simulink model "ASM_Traffic"  (R2026a)
settings: Solver=ode1  StartTime=SIM.tstart.v  StopTime=SIM.tend.v  FixedStep=SIM.StepSize.v
PostLoadFcn:
  | if any(exist('dsrtsu_mdlpostloadfcn', 'file') ~= 0), dsrtsu_mdlpostloadfcn('Execute', bdroot); end
  | try, asm_mdl_postloadfcn(bdroot, 'UpdateModel', 3600); catch, disp(lasterr); end,
InitFcn:
  | , if any(exist('rtifpga_mdlclblib', 'file') ~= 0), rtifpga_mdlclblib('Init', bdroot); end,
  | , if any(exist('dsmpb_private', 'file') ~= 0), dsmpb_private('dsmpb_mdlclblib', 'Init', bdroot); end,
model workspace (MAT data in the model file):
  asmReferencePath = [0 0.01 0.02 0.03 0.04 0.05 0.06 0.07 0.08 0.09 0.1 0.11 ... (350007 elements, 50001x7)]
  roadBounds : Simulink.Parameter (value not decoded)
  safetyAxes : Simulink.Parameter (value not decoded)
undefined symbols (not defined in the file): _to_, a0b2, ASM_BrakeHydraulics_DemoSystems, ASM_VehicleDynamics_DemoSystems, b98103fe8ad365046cd0, BrakeCircuit, controllerConfig, CPT, Crankshaft, DiscIntNeverNeededParam, dsmsi, FinalDriveAssembly, MDL, ModeSignals, mu, Pos_BrakePedal_Maneuver, rad, RefSignals, roadFamilyData, roadFamilyId, s_to_rpm, SIM, SoftECU, Suspension, Tire, Transmission
libraries: ASM_Traffic_lib x135, simulink x98, ASM_Utils_lib x77, ASM_VehicleDynamics_lib x70, ASM_Environment_lib x22, dsmpblib x20, dsmsilib x15, MDLD_Utils_lib x10, ASM_BrakeHydraulics_lib x3, sl_discontinuities x2
(part 49 of 65)

== system ASM_Traffic/Environment/Road/UserInterface/PAR_Plant/Objects_DataStreams/DataStream_5 ==
  Maneuver_Signals[] : Inport
  Bus Creator1 : BusCreator  Inputs=5
  Bus Selector2 : BusSelector  OutputSignals=Mnv_DataStream_5[]
  Ext_DataStream_5[] : Constant  Value=0
  Multiport Switch : MultiPortSwitch  DataPortOrder=Zero-based contiguous  zeroidx=on  SaturateOnIntegerOverflow=off  InputSameDT=off
  Rounding Function : Rounding  Operator=round
  Saturation : Saturate  UpperLimit=2  LowerLimit=0
  Stim_DataStream_5[] : Constant  Value=0
  Sw_DataStream_5[0Stim|1Ext|2Mnv] : Constant  Value=2
  avoid_incomplete_trace2source : Subsystem
  DataStream_5[] : Outport  VectorParamsAs1DForOutWhenUnconnected=off
  wires:
  avoid_incomplete_trace2source/1(Out1) -> Bus Creator1/3  "Mnv_DataStream_5[]"
  Sw_DataStream_5[0Stim|1Ext|2Mnv]/1 -> Rounding Function/1, Bus Creator1/1  "Sw_DataStream_5[0Stim|1Ext|2Mnv]"
  Maneuver_Signals[]/1 -> Bus Selector2/1
  Ext_DataStream_5[]/1 -> Multiport Switch/3, Bus Creator1/4  "Ext_DataStream_5[]"
  Bus Selector2/1 -> Multiport Switch/4, avoid_incomplete_trace2source/1(In1)  "<Mnv_DataStream_5[]>"
  Rounding Function/1 -> Saturation/1
  Saturation/1 -> Multiport Switch/1
  Multiport Switch/1 -> Bus Creator1/5  "DataStream_5[]"
  Stim_DataStream_5[]/1 -> Multiport Switch/2, Bus Creator1/2  "Stim_DataStream_5[]"
  Bus Creator1/1 -> DataStream_5[]/1

== system ASM_Traffic/Environment/Road/UserInterface/PAR_Plant/Objects_DataStreams/DataStream_6 ==
  Maneuver_Signals[] : Inport
  Bus Creator1 : BusCreator  Inputs=5
  Bus Selector2 : BusSelector  OutputSignals=Mnv_DataStream_6[]
  Ext_DataStream_6[] : Constant  Value=0
  Multiport Switch : MultiPortSwitch  DataPortOrder=Zero-based contiguous  zeroidx=on  SaturateOnIntegerOverflow=off  InputSameDT=off
  Rounding Function : Rounding  Operator=round
  Saturation : Saturate  UpperLimit=2  LowerLimit=0
  Stim_DataStream_6[] : Constant  Value=0
  Sw_DataStream_6[0Stim|1Ext|2Mnv] : Constant  Value=2
  avoid_incomplete_trace2source : Subsystem
  DataStream_6[] : Outport  VectorParamsAs1DForOutWhenUnconnected=off
  wires:
  avoid_incomplete_trace2source/1(Out1) -> Bus Creator1/3  "Mnv_DataStream_6[]"
  Bus Creator1/1 -> DataStream_6[]/1
  Stim_DataStream_6[]/1 -> Bus Creator1/2, Multiport Switch/2  "Stim_DataStream_6[]"
  Multiport Switch/1 -> Bus Creator1/5  "DataStream_6[]"
  Saturation/1 -> Multiport Switch/1
  Rounding Function/1 -> Saturation/1
  Bus Selector2/1 -> Multiport Switch/4, avoid_incomplete_trace2source/1(In1)  "<Mnv_DataStream_6[]>"
  Ext_DataStream_6[]/1 -> Multiport Switch/3, Bus Creator1/4  "Ext_DataStream_6[]"
  Maneuver_Signals[]/1 -> Bus Selector2/1
  Sw_DataStream_6[0Stim|1Ext|2Mnv]/1 -> Bus Creator1/1, Rounding Function/1  "Sw_DataStream_6[0Stim|1Ext|2Mnv]"

== system ASM_Traffic/Environment/Road/UserInterface/PAR_Plant/Objects_DataStreams/DataStream_7 ==
  Maneuver_Signals[] : Inport
  Bus Creator1 : BusCreator  Inputs=5
  Bus Selector2 : BusSelector  OutputSignals=Mnv_DataStream_7[]
  Ext_DataStream_7[] : Constant  Value=0
  Multiport Switch : MultiPortSwitch  DataPortOrder=Zero-based contiguous  zeroidx=on  SaturateOnIntegerOverflow=off  InputSameDT=off
  Rounding Function : Rounding  Operator=round
  Saturation : Saturate  UpperLimit=2  LowerLimit=0
  Stim_DataStream_7[] : Constant  Value=0
  Sw_DataStream_7[0Stim|1Ext|2Mnv] : Constant  Value=2
  avoid_incomplete_trace2source : Subsystem
  DataStream_7[] : Outport  VectorParamsAs1DForOutWhenUnconnected=off
  wires:
  avoid_incomplete_trace2source/1(Out1) -> Bus Creator1/3  "Mnv_DataStream_7[]"
  Sw_DataStream_7[0Stim|1Ext|2Mnv]/1 -> Rounding Function/1, Bus Creator1/1  "Sw_DataStream_7[0Stim|1Ext|2Mnv]"
  Maneuver_Signals[]/1 -> Bus Selector2/1
  Ext_DataStream_7[]/1 -> Multiport Switch/3, Bus Creator1/4  "Ext_DataStream_7[]"
  Bus Selector2/1 -> Multiport Switch/4, avoid_incomplete_trace2source/1(In1)  "<Mnv_DataStream_7[]>"
  Rounding Function/1 -> Saturation/1
  Saturation/1 -> Multiport Switch/1
  Multiport Switch/1 -> Bus Creator1/5  "DataStream_7[]"
  Stim_DataStream_7[]/1 -> Multiport Switch/2, Bus Creator1/2  "Stim_DataStream_7[]"
  Bus Creator1/1 -> DataStream_7[]/1

== system ASM_Traffic/Environment/Road/UserInterface/PAR_Plant/Objects_DataStreams/DataStream_8 ==
  Maneuver_Signals[] : Inport
  Bus Creator1 : BusCreator  Inputs=5
  Bus Selector2 : BusSelector  OutputSignals=Mnv_DataStream_8[]
  Ext_DataStream_8[] : Constant  Value=0
  Multiport Switch : MultiPortSwitch  DataPortOrder=Zero-based contiguous  zeroidx=on  SaturateOnIntegerOverflow=off  InputSameDT=off
  Rounding Function : Rounding  Operator=round
  Saturation : Saturate  UpperLimit=2  LowerLimit=0
  Stim_DataStream_8[] : Constant  Value=0
  Sw_DataStream_8[0Stim|1Ext|2Mnv] : Constant  Value=2
  avoid_incomplete_trace2source : Subsystem
  DataStream_8[] : Outport  VectorParamsAs1DForOutWhenUnconnected=off
  wires:
  avoid_incomplete_trace2source/1(Out1) -> Bus Creator1/3  "Mnv_DataStream_8[]"
  Bus Creator1/1 -> DataStream_8[]/1
  Stim_DataStream_8[]/1 -> Bus Creator1/2, Multiport Switch/2  "Stim_DataStream_8[]"
  Multiport Switch/1 -> Bus Creator1/5  "DataStream_8[]"
  Saturation/1 -> Multiport Switch/1
  Rounding Function/1 -> Saturation/1
  Bus Selector2/1 -> Multiport Switch/4, avoid_incomplete_trace2source/1(In1)  "<Mnv_DataStream_8[]>"
  Ext_DataStream_8[]/1 -> Multiport Switch/3, Bus Creator1/4  "Ext_DataStream_8[]"
  Maneuver_Signals[]/1 -> Bus Selector2/1
  Sw_DataStream_8[0Stim|1Ext|2Mnv]/1 -> Bus Creator1/1, Rounding Function/1  "Sw_DataStream_8[0Stim|1Ext|2Mnv]"

== system ASM_Traffic/Environment/Sensors/PlantModel/Object_Sensor_2D/ASMSignalCollector/Rename ==
  In1 : Inport
  Out1 : Outport  VectorParamsAs1DForOutWhenUnconnected=off
  wires:
  In1/1 -> Out1/1

== system ASM_Traffic/Environment/Sensors/PlantModel/Object_Sensor_2D/ASMSignalCollector/Rename1 ==
  In1 : Inport
  Out1 : Outport  VectorParamsAs1DForOutWhenUnconnected=off
  wires:
  In1/1 -> Out1/1

== system ASM_Traffic/Environment/Sensors/PlantModel/Object_Sensor_2D/ASMSignalCollector/Rename10 ==
  In1 : Inport
  Out1 : Outport  VectorParamsAs1DForOutWhenUnconnected=off
  wires:
  In1/1 -> Out1/1

== system ASM_Traffic/Environment/Sensors/PlantModel/Object_Sensor_2D/ASMSignalCollector/Rename11 ==
  In1 : Inport
  Out1 : Outport  VectorParamsAs1DForOutWhenUnconnected=off
  wires:
  In1/1 -> Out1/1

== system ASM_Traffic/Environment/Sensors/PlantModel/Object_Sensor_2D/ASMSignalCollector/Rename12 ==
  In1 : Inport
  Out1 : Outport  VectorParamsAs1DForOutWhenUnconnected=off
  wires:
  In1/1 -> Out1/1

== system ASM_Traffic/Environment/Sensors/PlantModel/Object_Sensor_2D/ASMSignalCollector/Rename13 ==
  In1 : Inport
  Out1 : Outport  VectorParamsAs1DForOutWhenUnconnected=off
  wires:
  In1/1 -> Out1/1

== system ASM_Traffic/Environment/Sensors/PlantModel/Object_Sensor_2D/ASMSignalCollector/Rename2 ==
  In1 : Inport
  Out1 : Outport  VectorParamsAs1DForOutWhenUnconnected=off
  wires:
  In1/1 -> Out1/1

== system ASM_Traffic/Environment/Sensors/PlantModel/Object_Sensor_2D/ASMSignalCollector/Rename3 ==
  In1 : Inport
  Out1 : Outport  VectorParamsAs1DForOutWhenUnconnected=off
  wires:
  In1/1 -> Out1/1

== system ASM_Traffic/Environment/Sensors/PlantModel/Object_Sensor_2D/ASMSignalCollector/Rename4 ==
  In1 : Inport
  Out1 : Outport  VectorParamsAs1DForOutWhenUnconnected=off
  wires:
  In1/1 -> Out1/1

== system ASM_Traffic/Environment/Sensors/PlantModel/Object_Sensor_2D/ASMSignalCollector/Rename5 ==
  In1 : Inport
  Out1 : Outport  VectorParamsAs1DForOutWhenUnconnected=off
  wires:
  In1/1 -> Out1/1

== system ASM_Traffic/Environment/Sensors/PlantModel/Object_Sensor_2D/ASMSignalCollector/Rename6 ==
  In1 : Inport
  Out1 : Outport  VectorParamsAs1DForOutWhenUnconnected=off
  wires:
  In1/1 -> Out1/1

== system ASM_Traffic/Environment/Sensors/PlantModel/Object_Sensor_2D/ASMSignalCollector/Rename7 ==
  In1 : Inport
  Out1 : Outport  VectorParamsAs1DForOutWhenUnconnected=off
  wires:
  In1/1 -> Out1/1

== system ASM_Traffic/Environment/Sensors/PlantModel/Object_Sensor_2D/ASMSignalCollector/Rename8 ==
  In1 : Inport
  Out1 : Outport  VectorParamsAs1DForOutWhenUnconnected=off
  wires:
  In1/1 -> Out1/1

== system ASM_Traffic/Environment/Sensors/PlantModel/Object_Sensor_2D/ASMSignalCollector/Rename9 ==
  In1 : Inport
  Out1 : Outport  VectorParamsAs1DForOutWhenUnconnected=off
  wires:
  In1/1 -> Out1/1

== system ASM_Traffic/Environment/Sensors/PlantModel/Object_Sensor_2D/ObjectData/Sensor1 ==
  Object_ID[] : Inport
  Object_Type[] : Inport  Port=2
  Traffic_Signals : Inport  Port=3
  Road_Signals : Inport  Port=4
  ASMSignalCollector : Subsystem
  Bus Selector4 : BusSelector  OutputSignals=Plant.Road_TrafficFellows.Network_Item_Type_Fellows[],Plant.Road_TrafficFellows.Network_Item_Id_Fellows[],Plant.TrafficObject_Data[]
  Bus Selector5 : BusSelector  OutputSignals=Plant.Traffic_Signals_toEnvironment
  Bus Selector6 : BusSelector  OutputSignals=Plant.ObjectParameters.TrafficObjects.TrafficObject_Type_Data[]
  GetFellowPositionVector : Subsystem
  OBJECT_POSITION : ASM_Traffic_lib/Objects/OBJECT_POSITION  MaxNumFellows=MDL.Traffic.MaxNumFellows  ASMProperties=struct('Name','OBJECT_POSITION','Version','2.0','Library','ASM_Traffic_lib')  ASMInstanceName=object_position  ASMInstanceID=1
  OBJECT_PROPERTIES_BOX : ASM_Traffic_lib/Objects/OBJECT_PROPERTIES_BOX  ASMProperties=struct('Name','OBJECT_PROPERTIES_BOX','Version','2.0','Library','ASM_Traffic_lib')  ASMInstanceName=object_properties_box  ASMInstanceID=1
  Object_Custom_Values : Subsystem
  Terminator : Terminator
  Terminator1 : Terminator
  ASMSignalBus : Outport  VectorParamsAs1DForOutWhenUnconnected=off
  Object_Position[] : Outport  Port=2  VectorParamsAs1DForOutWhenUnconnected=off
  Object_Properties_Box[] : Outport  Port=3  VectorParamsAs1DForOutWhenUnconnected=off
  Object_Custom_Values[] : Outport  Port=4  VectorParamsAs1DForOutWhenUnconnected=off
  wires:
  Bus Selector5/1 -> GetFellowPositionVector/1(<FellowPositions>)  "<Traffic_Signals_toEnvironment>"
  GetFellowPositionVector/2(Angle_Fellows[deg]) -> OBJECT_POSITION/3
  GetFellowPositionVector/1(Pos_Fellows_MainPnt_CoorSys_E[x;y;z][m]) -> OBJECT_POSITION/2
  OBJECT_PROPERTIES_BOX/2 -> Object_Properties_Box[]/1, ASMSignalCollector/2(Object_Properties_Box)
  ASMSignalCollector/1(ASMSignalBus) -> ASMSignalBus/1
  OBJECT_POSITION/2 -> Object_Position[]/1, ASMSignalCollector/1(Object_Positions)
  Object_Custom_Values/1(Object_Custom_Values[]) -> ASMSignalCollector/3(Object_Custom_Values), Object_Custom_Values[]/1  "Object_Custom_Values"
  Bus Selector6/1 -> Object_Custom_Values/2(TrafficObject_Type_Data[]), OBJECT_PROPERTIES_BOX/2  "<TrafficObject_Type_Data[]>"
  Traffic_Signals/1 -> Bus Selector6/1, Bus Selector5/1
  Bus Selector4/3 -> OBJECT_POSITION/6  "<TrafficObject_Data[]>"
  Bus Selector4/2 -> OBJECT_POSITION/5  "<Network_Item_Id_Fellows[]>"
  Bus Selector4/1 -> OBJECT_POSITION/4  "<Network_Item_Type_Fellows[]>"
  Road_Signals/1 -> Bus Selector4/1
  Object_Type[]/1 -> OBJECT_PROPERTIES_BOX/1, Object_Custom_Values/1(TrafficObject_Type[])
  OBJECT_PROPERTIES_BOX/1 -> Terminator1/1
  Object_ID[]/1 -> OBJECT_POSITION/1
  OBJECT_POSITION/1 -> Terminator/1

== system ASM_Traffic/Environment/Sensors/PlantModel/Object_Sensor_2D/ObjectData/Sensor2 ==
  Object_ID[] : Inport
  Object_Type[] : Inport  Port=2
  Traffic_Signals : Inport  Port=3
  Road_Signals : Inport  Port=4
  ASMSignalCollector : Subsystem
  Bus Selector4 : BusSelector  OutputSignals=Plant.Road_TrafficFellows.Network_Item_Type_Fellows[],Plant.Road_TrafficFellows.Network_Item_Id_Fellows[],Plant.TrafficObject_Data[]
  Bus Selector5 : BusSelector  OutputSignals=Plant.Traffic_Signals_toEnvironment
  Bus Selector6 : BusSelector  OutputSignals=Plant.ObjectParameters.TrafficObjects.TrafficObject_Type_Data[]
  GetFellowPositionVector : Subsystem
  OBJECT_POSITION : ASM_Traffic_lib/Objects/OBJECT_POSITION  MaxNumFellows=MDL.Traffic.MaxNumFellows  ASMProperties=struct('Name','OBJECT_POSITION','Version','2.0','Library','ASM_Traffic_lib')  ASMInstanceName=object_position  ASMInstanceID=1
  OBJECT_PROPERTIES_BOX : ASM_Traffic_lib/Objects/OBJECT_PROPERTIES_BOX  ASMProperties=struct('Name','OBJECT_PROPERTIES_BOX','Version','2.0','Library','ASM_Traffic_lib')  ASMInstanceName=object_properties_box  ASMInstanceID=1
  Object_Custom_Values : Subsystem
  Terminator : Terminator
  Terminator1 : Terminator
  ASMSignalBus : Outport  VectorParamsAs1DForOutWhenUnconnected=off
  Object_Position[] : Outport  Port=2  VectorParamsAs1DForOutWhenUnconnected=off
  Object_Properties_Box[] : Outport  Port=3  VectorParamsAs1DForOutWhenUnconnected=off
  Object_Custom_Values[] : Outport  Port=4  VectorParamsAs1DForOutWhenUnconnected=off
  wires:
  GetFellowPositionVector/1(Pos_Fellows_MainPnt_CoorSys_E[x;y;z][m]) -> OBJECT_POSITION/2
  GetFellowPositionVector/2(Angle_Fellows[deg]) -> OBJECT_POSITION/3
  Traffic_Signals/1 -> Bus Selector6/1, Bus Selector5/1
  Bus Selector5/1 -> GetFellowPositionVector/1(<FellowPositions>)  "<Traffic_Signals_toEnvironment>"
  Object_Custom_Values/1(Object_Custom_Values[]) -> Object_Custom_Values[]/1, ASMSignalCollector/3(Object_Custom_Values)  "Object_Custom_Values"
  OBJECT_POSITION/2 -> Object_Position[]/1, ASMSignalCollector/1(Object_Positions)
  OBJECT_PROPERTIES_BOX/2 -> Object_Properties_Box[]/1, ASMSignalCollector/2(Object_Properties_Box)
  ASMSignalCollector/1(ASMSignalBus) -> ASMSignalBus/1
  OBJECT_POSITION/1 -> Terminator/1
  Object_ID[]/1 -> OBJECT_POSITION/1
  OBJECT_PROPERTIES_BOX/1 -> Terminator1/1
  Object_Type[]/1 -> Object_Custom_Values/1(TrafficObject_Type[]), OBJECT_PROPERTIES_BOX/1
  Road_Signals/1 -> Bus Selector4/1
  Bus Selector4/1 -> OBJECT_POSITION/4  "<Network_Item_Type_Fellows[]>"
  Bus Selector4/2 -> OBJECT_POSITION/5  "<Network_Item_Id_Fellows[]>"
  Bus Selector4/3 -> OBJECT_POSITION/6  "<TrafficObject_Data[]>"
  Bus Selector6/1 -> Object_Custom_Values/2(TrafficObject_Type_Data[]), OBJECT_PROPERTIES_BOX/2  "<TrafficObject_Type_Data[]>"

== system ASM_Traffic/Environment/Sensors/PlantModel/Object_Sensor_2D/ObjectData/Sensor3 ==
  Object_ID[] : Inport
  Object_Type[] : Inport  Port=2
  Traffic_Signals : Inport  Port=3
  Road_Signals : Inport  Port=4
  ASMSignalCollector : Subsystem
  Bus Selector4 : BusSelector  OutputSignals=Plant.Road_TrafficFellows.Network_Item_Type_Fellows[],Plant.Road_TrafficFellows.Network_Item_Id_Fellows[],Plant.TrafficObject_Data[]
  Bus Selector5 : BusSelector  OutputSignals=Plant.Traffic_Signals_toEnvironment
  Bus Selector6 : BusSelector  OutputSignals=Plant.ObjectParameters.TrafficObjects.TrafficObject_Type_Data[]
  GetFellowPositionVector : Subsystem
  OBJECT_POSITION : ASM_Traffic_lib/Objects/OBJECT_POSITION  MaxNumFellows=MDL.Traffic.MaxNumFellows  ASMProperties=struct('Name','OBJECT_POSITION','Version','2.0','Library','ASM_Traffic_lib')  ASMInstanceName=object_position  ASMInstanceID=1
  OBJECT_PROPERTIES_BOX : ASM_Traffic_lib/Objects/OBJECT_PROPERTIES_BOX  ASMProperties=struct('Name','OBJECT_PROPERTIES_BOX','Version','2.0','Library','ASM_Traffic_lib')  ASMInstanceName=object_properties_box  ASMInstanceID=1
  Object_Custom_Values : Subsystem
  Terminator : Terminator
  Terminator1 : Terminator
  ASMSignalBus : Outport  VectorParamsAs1DForOutWhenUnconnected=off
  Object_Position[] : Outport  Port=2  VectorParamsAs1DForOutWhenUnconnected=off
  Object_Properties_Box[] : Outport  Port=3  VectorParamsAs1DForOutWhenUnconnected=off
  Object_Custom_Values[] : Outport  Port=4  VectorParamsAs1DForOutWhenUnconnected=off
  wires:
  GetFellowPositionVector/1(Pos_Fellows_MainPnt_CoorSys_E[x;y;z][m]) -> OBJECT_POSITION/2
  GetFellowPositionVector/2(Angle_Fellows[deg]) -> OBJECT_POSITION/3
  Traffic_Signals/1 -> Bus Selector6/1, Bus Selector5/1
  Bus Selector5/1 -> GetFellowPositionVector/1(<FellowPositions>)  "<Traffic_Signals_toEnvironment>"
  Object_Custom_Values/1(Object_Custom_Values[]) -> Object_Custom_Values[]/1, ASMSignalCollector/3(Object_Custom_Values)  "Object_Custom_Values"
  OBJECT_POSITION/2 -> Object_Position[]/1, ASMSignalCollector/1(Object_Positions)
  OBJECT_PROPERTIES_BOX/2 -> Object_Properties_Box[]/1, ASMSignalCollector/2(Object_Properties_Box)
  ASMSignalCollector/1(ASMSignalBus) -> ASMSignalBus/1
  Bus Selector6/1 -> Object_Custom_Values/2(TrafficObject_Type_Data[]), OBJECT_PROPERTIES_BOX/2  "<TrafficObject_Type_Data[]>"
  Bus Selector4/3 -> OBJECT_POSITION/6  "<TrafficObject_Data[]>"
  Bus Selector4/2 -> OBJECT_POSITION/5  "<Network_Item_Id_Fellows[]>"
  Bus Selector4/1 -> OBJECT_POSITION/4  "<Network_Item_Type_Fellows[]>"
  Road_Signals/1 -> Bus Selector4/1
  Object_Type[]/1 -> Object_Custom_Values/1(TrafficObject_Type[]), OBJECT_PROPERTIES_BOX/1
  OBJECT_PROPERTIES_BOX/1 -> Terminator1/1
  Object_ID[]/1 -> OBJECT_POSITION/1
  OBJECT_POSITION/1 -> Terminator/1

== system ASM_Traffic/Environment/Sensors/PlantModel/Object_Sensor_2D/ObjectData/Sensor4 ==
  Object_ID[] : Inport
  Object_Type[] : Inport  Port=2
  Traffic_Signals : Inport  Port=3
  Road_Signals : Inport  Port=4
  ASMSignalCollector : Subsystem
  Bus Selector1 : BusSelector  OutputSignals=Plant.Traffic_Signals_toEnvironment
  Bus Selector4 : BusSelector  OutputSignals=Plant.Road_TrafficFellows.Network_Item_Type_Fellows[],Plant.Road_TrafficFellows.Network_Item_Id_Fellows[],Plant.TrafficObject_Data[]
  Bus Selector6 : BusSelector  OutputSignals=Plant.ObjectParameters.TrafficObjects.TrafficObject_Type_Data[]
  GetFellowPositionVector : Subsystem
  OBJECT_POSITION : ASM_Traffic_lib/Objects/OBJECT_POSITION  MaxNumFellows=MDL.Traffic.MaxNumFellows  ASMProperties=struct('Name','OBJECT_POSITION','Version','2.0','Library','ASM_Traffic_lib')  ASMInstanceName=object_position  ASMInstanceID=1
  OBJECT_PROPERTIES_BOX : ASM_Traffic_lib/Objects/OBJECT_PROPERTIES_BOX  ASMProperties=struct('Name','OBJECT_PROPERTIES_BOX','Version','2.0','Library','ASM_Traffic_lib')  ASMInstanceName=object_properties_box  ASMInstanceID=1
  Object_Custom_Values : Subsystem
  Terminator : Terminator
  Terminator1 : Terminator
  ASMSignalBus : Outport  VectorParamsAs1DForOutWhenUnconnected=off
  Object_Position[] : Outport  Port=2  VectorParamsAs1DForOutWhenUnconnected=off
  Object_Properties_Box[] : Outport  Port=3  VectorParamsAs1DForOutWhenUnconnected=off
  Object_Custom_Values[] : Outport  Port=4  VectorParamsAs1DForOutWhenUnconnected=off
  wires:
  Traffic_Signals/1 -> Bus Selector6/1, Bus Selector1/1
  GetFellowPositionVector/1(Pos_Fellows_MainPnt_CoorSys_E[x;y;z][m]) -> OBJECT_POSITION/2
  GetFellowPositionVector/2(Angle_Fellows[deg]) -> OBJECT_POSITION/3
  Bus Selector1/1 -> GetFellowPositionVector/1(<FellowPositions>)  "<Traffic_Signals_toEnvironment>"
  Object_Custom_Values/1(Object_Custom_Values[]) -> Object_Custom_Values[]/1, ASMSignalCollector/3(Object_Custom_Values)  "Object_Custom_Values"
  OBJECT_POSITION/2 -> Object_Position[]/1, ASMSignalCollector/1(Object_Positions)
  OBJECT_PROPERTIES_BOX/2 -> Object_Properties_Box[]/1, ASMSignalCollector/2(Object_Properties_Box)
  ASMSignalCollector/1(ASMSignalBus) -> ASMSignalBus/1
  Bus Selector6/1 -> Object_Custom_Values/2(TrafficObject_Type_Data[]), OBJECT_PROPERTIES_BOX/2  "<TrafficObject_Type_Data[]>"
  Bus Selector4/3 -> OBJECT_POSITION/6  "<TrafficObject_Data[]>"
  Bus Selector4/2 -> OBJECT_POSITION/5  "<Network_Item_Id_Fellows[]>"
  Bus Selector4/1 -> OBJECT_POSITION/4  "<Network_Item_Type_Fellows[]>"
  Road_Signals/1 -> Bus Selector4/1
  Object_Type[]/1 -> Object_Custom_Values/1(TrafficObject_Type[]), OBJECT_PROPERTIES_BOX/1
  OBJECT_PROPERTIES_BOX/1 -> Terminator1/1
  Object_ID[]/1 -> OBJECT_POSITION/1
  OBJECT_POSITION/1 -> Terminator/1

== system ASM_Traffic/Environment/Sensors/PlantModel/Object_Sensor_2D/ObjectData/Sensor5 ==
  Object_ID[] : Inport
  Object_Type[] : Inport  Port=2
  Traffic_Signals : Inport  Port=3
  Road_Signals : Inport  Port=4
  ASMSignalCollector : Subsystem
  Bus Selector4 : BusSelector  OutputSignals=Plant.Road_TrafficFellows.Network_Item_Type_Fellows[],Plant.Road_TrafficFellows.Network_Item_Id_Fellows[],Plant.TrafficObject_Data[]
  Bus Selector5 : BusSelector  OutputSignals=Plant.Traffic_Signals_toEnvironment
  Bus Selector6 : BusSelector  OutputSignals=Plant.ObjectParameters.TrafficObjects.TrafficObject_Type_Data[]
  GetFellowPositionVector : Subsystem
  OBJECT_POSITION : ASM_Traffic_lib/Objects/OBJECT_POSITION  MaxNumFellows=MDL.Traffic.MaxNumFellows  ASMProperties=struct('Name','OBJECT_POSITION','Version','2.0','Library','ASM_Traffic_lib')  ASMInstanceName=object_position  ASMInstanceID=1
  OBJECT_PROPERTIES_BOX : ASM_Traffic_lib/Objects/OBJECT_PROPERTIES_BOX  ASMProperties=struct('Name','OBJECT_PROPERTIES_BOX','Version','2.0','Library','ASM_Traffic_lib')  ASMInstanceName=object_properties_box  ASMInstanceID=1
  Object_Custom_Values : Subsystem
  Terminator : Terminator
  Terminator1 : Terminator
  ASMSignalBus : Outport  VectorParamsAs1DForOutWhenUnconnected=off
  Object_Position[] : Outport  Port=2  VectorParamsAs1DForOutWhenUnconnected=off
  Object_Properties_Box[] : Outport  Port=3  VectorParamsAs1DForOutWhenUnconnected=off
  Object_Custom_Values[] : Outport  Port=4  VectorParamsAs1DForOutWhenUnconnected=off
  wires:
  GetFellowPositionVector/1(Pos_Fellows_MainPnt_CoorSys_E[x;y;z][m]) -> OBJECT_POSITION/2
  GetFellowPositionVector/2(Angle_Fellows[deg]) -> OBJECT_POSITION/3
  Traffic_Signals/1 -> Bus Selector6/1, Bus Selector5/1
  Bus Selector5/1 -> GetFellowPositionVector/1(<FellowPositions>)  "<Traffic_Signals_toEnvironment>"
  Object_Custom_Values/1(Object_Custom_Values[]) -> Object_Custom_Values[]/1, ASMSignalCollector/3(Object_Custom_Values)  "Object_Custom_Values"
  OBJECT_POSITION/2 -> Object_Position[]/1, ASMSignalCollector/1(Object_Positions)
  OBJECT_PROPERTIES_BOX/2 -> Object_Properties_Box[]/1, ASMSignalCollector/2(Object_Properties_Box)
  ASMSignalCollector/1(ASMSignalBus) -> ASMSignalBus/1
  OBJECT_POSITION/1 -> Terminator/1
  Object_ID[]/1 -> OBJECT_POSITION/1
  OBJECT_PROPERTIES_BOX/1 -> Terminator1/1
  Object_Type[]/1 -> Object_Custom_Values/1(TrafficObject_Type[]), OBJECT_PROPERTIES_BOX/1
  Road_Signals/1 -> Bus Selector4/1
  Bus Selector4/1 -> OBJECT_POSITION/4  "<Network_Item_Type_Fellows[]>"
  Bus Selector4/2 -> OBJECT_POSITION/5  "<Network_Item_Id_Fellows[]>"
  Bus Selector4/3 -> OBJECT_POSITION/6  "<TrafficObject_Data[]>"
  Bus Selector6/1 -> Object_Custom_Values/2(TrafficObject_Type_Data[]), OBJECT_PROPERTIES_BOX/2  "<TrafficObject_Type_Data[]>"

== system ASM_Traffic/Environment/Sensors/PlantModel/Object_Sensor_2D/ObjectData/Sensor6 ==
  Object_ID[] : Inport
  Object_Type[] : Inport  Port=2
  Traffic_Signals : Inport  Port=3
  Road_Signals : Inport  Port=4
  ASMSignalCollector : Subsystem
  Bus Selector4 : BusSelector  OutputSignals=Plant.Road_TrafficFellows.Network_Item_Type_Fellows[],Plant.Road_TrafficFellows.Network_Item_Id_Fellows[],Plant.TrafficObject_Data[]
  Bus Selector5 : BusSelector  OutputSignals=Plant.Traffic_Signals_toEnvironment
  Bus Selector6 : BusSelector  OutputSignals=Plant.ObjectParameters.TrafficObjects.TrafficObject_Type_Data[]
  GetFellowPositionVector : Subsystem
  OBJECT_POSITION : ASM_Traffic_lib/Objects/OBJECT_POSITION  MaxNumFellows=MDL.Traffic.MaxNumFellows  ASMProperties=struct('Name','OBJECT_POSITION','Version','2.0','Library','ASM_Traffic_lib')  ASMInstanceName=object_position  ASMInstanceID=1
  OBJECT_PROPERTIES_BOX : ASM_Traffic_lib/Objects/OBJECT_PROPERTIES_BOX  ASMProperties=struct('Name','OBJECT_PROPERTIES_BOX','Version','2.0','Library','ASM_Traffic_lib')  ASMInstanceName=object_properties_box  ASMInstanceID=1
  Object_Custom_Values : Subsystem
  Terminator : Terminator
  Terminator1 : Terminator
  ASMSignalBus : Outport  VectorParamsAs1DForOutWhenUnconnected=off
  Object_Position[] : Outport  Port=2  VectorParamsAs1DForOutWhenUnconnected=off
  Object_Properties_Box[] : Outport  Port=3  VectorParamsAs1DForOutWhenUnconnected=off
  Object_Custom_Values[] : Outport  Port=4  VectorParamsAs1DForOutWhenUnconnected=off
  wires:
  Traffic_Signals/1 -> Bus Selector6/1, Bus Selector5/1
  Bus Selector5/1 -> GetFellowPositionVector/1(<FellowPositions>)  "<Traffic_Signals_toEnvironment>"
  GetFellowPositionVector/1(Pos_Fellows_MainPnt_CoorSys_E[x;y;z][m]) -> OBJECT_POSITION/2
  GetFellowPositionVector/2(Angle_Fellows[deg]) -> OBJECT_POSITION/3
  Object_Custom_Values/1(Object_Custom_Values[]) -> Object_Custom_Values[]/1, ASMSignalCollector/3(Object_Custom_Values)  "Object_Custom_Values"
  OBJECT_POSITION/2 -> Object_Position[]/1, ASMSignalCollector/1(Object_Positions)
  OBJECT_PROPERTIES_BOX/2 -> Object_Properties_Box[]/1, ASMSignalCollector/2(Object_Properties_Box)
  ASMSignalCollector/1(ASMSignalBus) -> ASMSignalBus/1
  Bus Selector6/1 -> Object_Custom_Values/2(TrafficObject_Type_Data[]), OBJECT_PROPERTIES_BOX/2  "<TrafficObject_Type_Data[]>"
  Bus Selector4/3 -> OBJECT_POSITION/6  "<TrafficObject_Data[]>"
  Bus Selector4/2 -> OBJECT_POSITION/5  "<Network_Item_Id_Fellows[]>"
  Bus Selector4/1 -> OBJECT_POSITION/4  "<Network_Item_Type_Fellows[]>"
  Road_Signals/1 -> Bus Selector4/1
  Object_Type[]/1 -> Object_Custom_Values/1(TrafficObject_Type[]), OBJECT_PROPERTIES_BOX/1
  OBJECT_PROPERTIES_BOX/1 -> Terminator1/1
  Object_ID[]/1 -> OBJECT_POSITION/1
  OBJECT_POSITION/1 -> Terminator/1

== system ASM_Traffic/Environment/Sensors/PlantModel/Object_Sensor_2D/ObjectData/Sensor7 ==
  Object_ID[] : Inport
  Object_Type[] : Inport  Port=2
  Traffic_Signals : Inport  Port=3
  Road_Signals : Inport  Port=4
  ASMSignalCollector : Subsystem
  Bus Selector4 : BusSelector  OutputSignals=Plant.Road_TrafficFellows.Network_Item_Type_Fellows[],Plant.Road_TrafficFellows.Network_Item_Id_Fellows[],Plant.TrafficObject_Data[]
  Bus Selector5 : BusSelector  OutputSignals=Plant.Traffic_Signals_toEnvironment
  Bus Selector6 : BusSelector  OutputSignals=Plant.ObjectParameters.TrafficObjects.TrafficObject_Type_Data[]
  GetFellowPositionVector : Subsystem
  OBJECT_POSITION : ASM_Traffic_lib/Objects/OBJECT_POSITION  MaxNumFellows=MDL.Traffic.MaxNumFellows  ASMProperties=struct('Name','OBJECT_POSITION','Version','2.0','Library','ASM_Traffic_lib')  ASMInstanceName=object_position  ASMInstanceID=1
  OBJECT_PROPERTIES_BOX : ASM_Traffic_lib/Objects/OBJECT_PROPERTIES_BOX  ASMProperties=struct('Name','OBJECT_PROPERTIES_BOX','Version','2.0','Library','ASM_Traffic_lib')  ASMInstanceName=object_properties_box  ASMInstanceID=1
  Object_Custom_Values : Subsystem
  Terminator : Terminator
  Terminator1 : Terminator
  ASMSignalBus : Outport  VectorParamsAs1DForOutWhenUnconnected=off
  Object_Position[] : Outport  Port=2  VectorParamsAs1DForOutWhenUnconnected=off
  Object_Properties_Box[] : Outport  Port=3  VectorParamsAs1DForOutWhenUnconnected=off
  Object_Custom_Values[] : Outport  Port=4  VectorParamsAs1DForOutWhenUnconnected=off
  wires:
  Traffic_Signals/1 -> Bus Selector6/1, Bus Selector5/1
  Bus Selector5/1 -> GetFellowPositionVector/1(<FellowPositions>)  "<Traffic_Signals_toEnvironment>"
  GetFellowPositionVector/1(Pos_Fellows_MainPnt_CoorSys_E[x;y;z][m]) -> OBJECT_POSITION/2
  GetFellowPositionVector/2(Angle_Fellows[deg]) -> OBJECT_POSITION/3
  Object_Custom_Values/1(Object_Custom_Values[]) -> Object_Custom_Values[]/1, ASMSignalCollector/3(Object_Custom_Values)  "Object_Custom_Values"
  OBJECT_POSITION/2 -> Object_Position[]/1, ASMSignalCollector/1(Object_Positions)
  OBJECT_PROPERTIES_BOX/2 -> Object_Properties_Box[]/1, ASMSignalCollector/2(Object_Properties_Box)
  ASMSignalCollector/1(ASMSignalBus) -> ASMSignalBus/1
  OBJECT_POSITION/1 -> Terminator/1
  Object_ID[]/1 -> OBJECT_POSITION/1
  OBJECT_PROPERTIES_BOX/1 -> Terminator1/1
  Object_Type[]/1 -> Object_Custom_Values/1(TrafficObject_Type[]), OBJECT_PROPERTIES_BOX/1
  Road_Signals/1 -> Bus Selector4/1
  Bus Selector4/1 -> OBJECT_POSITION/4  "<Network_Item_Type_Fellows[]>"
  Bus Selector4/2 -> OBJECT_POSITION/5  "<Network_Item_Id_Fellows[]>"
  Bus Selector4/3 -> OBJECT_POSITION/6  "<TrafficObject_Data[]>"
  Bus Selector6/1 -> Object_Custom_Values/2(TrafficObject_Type_Data[]), OBJECT_PROPERTIES_BOX/2  "<TrafficObject_Type_Data[]>"

== system ASM_Traffic/Environment/Sensors/PlantModel/Object_Sensor_2D/ObjectData/avoid_incomplete_trace2source ==
  In1 : Inport
  DummyGain : Gain
  Out1 : Outport
  wires:
  In1/1 -> DummyGain/1
  DummyGain/1 -> Out1/1

== system ASM_Traffic/Environment/Sensors/PlantModel/Object_Sensor_2D/ObjectData/avoid_incomplete_trace2source1 ==
  In1 : Inport
  DummyGain : Gain
  Out1 : Outport
  wires:
  DummyGain/1 -> Out1/1
  In1/1 -> DummyGain/1

== system ASM_Traffic/Environment/Sensors/PlantModel/Object_Sensor_2D/ObjectData/avoid_incomplete_trace2source10 ==
  In1 : Inport
  DummyGain : Gain
  Out1 : Outport
  wires:
  DummyGain/1 -> Out1/1
  In1/1 -> DummyGain/1

== system ASM_Traffic/Environment/Sensors/PlantModel/Object_Sensor_2D/ObjectData/avoid_incomplete_trace2source11 ==
  In1 : Inport
  DummyGain : Gain
  Out1 : Outport
  wires:
  In1/1 -> DummyGain/1
  DummyGain/1 -> Out1/1

== system ASM_Traffic/Environment/Sensors/PlantModel/Object_Sensor_2D/ObjectData/avoid_incomplete_trace2source12 ==
  In1 : Inport
  DummyGain : Gain
  Out1 : Outport
  wires:
  In1/1 -> DummyGain/1
  DummyGain/1 -> Out1/1

== system ASM_Traffic/Environment/Sensors/PlantModel/Object_Sensor_2D/ObjectData/avoid_incomplete_trace2source13 ==
  In1 : Inport
  DummyGain : Gain
  Out1 : Outport
  wires:
  DummyGain/1 -> Out1/1
  In1/1 -> DummyGain/1

== system ASM_Traffic/Environment/Sensors/PlantModel/Object_Sensor_2D/ObjectData/avoid_incomplete_trace2source2 ==
  In1 : Inport
  DummyGain : Gain
  Out1 : Outport
  wires:
  DummyGain/1 -> Out1/1
  In1/1 -> DummyGain/1

== system ASM_Traffic/Environment/Sensors/PlantModel/Object_Sensor_2D/ObjectData/avoid_incomplete_trace2source3 ==
  In1 : Inport
  DummyGain : Gain
  Out1 : Outport
  wires:
  In1/1 -> DummyGain/1
  DummyGain/1 -> Out1/1

== system ASM_Traffic/Environment/Sensors/PlantModel/Object_Sensor_2D/ObjectData/avoid_incomplete_trace2source4 ==
  In1 : Inport
  DummyGain : Gain
  Out1 : Outport
  wires:
  In1/1 -> DummyGain/1
  DummyGain/1 -> Out1/1

== system ASM_Traffic/Environment/Sensors/PlantModel/Object_Sensor_2D/ObjectData/avoid_incomplete_trace2source5 ==
  In1 : Inport
  DummyGain : Gain
  Out1 : Outport
  wires:
  DummyGain/1 -> Out1/1
  In1/1 -> DummyGain/1

== system ASM_Traffic/Environment/Sensors/PlantModel/Object_Sensor_2D/ObjectData/avoid_incomplete_trace2source6 ==
  In1 : Inport
  DummyGain : Gain
  Out1 : Outport
  wires:
  DummyGain/1 -> Out1/1
  In1/1 -> DummyGain/1

== system ASM_Traffic/Environment/Sensors/PlantModel/Object_Sensor_2D/ObjectData/avoid_incomplete_trace2source7 ==
  In1 : Inport
  DummyGain : Gain
  Out1 : Outport
  wires:
  In1/1 -> DummyGain/1
  DummyGain/1 -> Out1/1

== system ASM_Traffic/Environment/Sensors/PlantModel/Object_Sensor_2D/ObjectData/avoid_incomplete_trace2source8 ==
  In1 : Inport
  DummyGain : Gain
  Out1 : Outport
  wires:
  In1/1 -> DummyGain/1
  DummyGain/1 -> Out1/1

== system ASM_Traffic/Environment/Sensors/PlantModel/Object_Sensor_2D/ObjectData/avoid_incomplete_trace2source9 ==
  In1 : Inport
  DummyGain : Gain
  Out1 : Outport
  wires:
  DummyGain/1 -> Out1/1
  In1/1 -> DummyGain/1

== system ASM_Traffic/Environment/Sensors/PlantModel/Object_Sensor_2D/ScheduleAndCalculateSensor/GetFellowPositionVector ==
  <FellowPositions> : Inport
  Bus Selector11 : BusSelector  OutputSignals=Pos_Fellows_MainPnt_CoorSys_E[x;y;z][m].Pos_x_Fellows[m],Pos_Fellows_MainPnt_CoorSys_E[x;y;z][m].Pos_y_Fellows[m],Pos_Fellows_MainPnt_CoorSys_E[x;y;z][m].Pos_z_Fellows[m],Angle_Fellows[x;y;z][deg].Angle_Roll_Fellows[deg],Angle_Fellows[x;y;z][deg].Angle_Pitch_Fellows[deg],Angle_Fellows[x;y;z][deg].Angle_Yaw_Fellows[deg]
  Mux1 : Mux  Inputs=3
  Mux2 : Mux  Inputs=3
  Pos_Fellows_MainPnt_CoorSys_E[x;y;z][m] : Outport  VectorParamsAs1DForOutWhenUnconnected=off
  Angle_Fellows[deg] : Outport  Port=2  VectorParamsAs1DForOutWhenUnconnected=off
  wires:
  Mux2/1 -> Pos_Fellows_MainPnt_CoorSys_E[x;y;z][m]/1  "Pos_Fellows_MainPnt_CoorSys_E[x;y;z][m]"
  Mux1/1 -> Angle_Fellows[deg]/1  "Pos_Fellows_MainPnt_CoorSys_E_vec"
  Bus Selector11/4 -> Mux1/1  "<Angle_Roll_Fellows[deg]>"
  Bus Selector11/1 -> Mux2/1  "<Pos_x_Fellows[m]>"
  Bus Selector11/2 -> Mux2/2  "<Pos_y_Fellows[m]>"
  Bus Selector11/6 -> Mux1/3  "<Angle_Yaw_Fellows[deg]>"
  Bus Selector11/5 -> Mux1/2  "<Angle_Pitch_Fellows[deg]>"
  <FellowPositions>/1 -> Bus Selector11/1
  Bus Selector11/3 -> Mux2/3  "<Pos_z_Fellows[m]>"

== system ASM_Traffic/Environment/Sensors/PlantModel/Object_Sensor_2D/ScheduleAndCalculateSensor/SampleAndHold ==
  In1 : Inport
  In2 : Inport  Port=2
  In3 : Inport  Port=3
  In4 : Inport  Port=4
  In5 : Inport  Port=5
  Enable : EnablePort
  Out1 : Outport  VectorParamsAs1DForOutWhenUnconnected=off
  Out2 : Outport  Port=2  VectorParamsAs1DForOutWhenUnconnected=off
  Out3 : Outport  Port=3  VectorParamsAs1DForOutWhenUnconnected=off
  Out4 : Outport  Port=4  VectorParamsAs1DForOutWhenUnconnected=off
  Out5 : Outport  Port=5  VectorParamsAs1DForOutWhenUnconnected=off
  wires:
  In5/1 -> Out5/1
  In4/1 -> Out4/1
  In3/1 -> Out3/1
  In1/1 -> Out1/1
  In2/1 -> Out2/1

== system ASM_Traffic/Environment/Sensors/PlantModel/Object_Sensor_2D/SensorParameters/2D_Sensors_Common_Signals ==
  Sensor_Data[] : Inport
  Bus Creator1 : BusCreator  Inputs=1
  Compare To Constant : simulink/Logic and Bit Operations/Compare To Constant  relop===  const=1  OutDataTypeStr=boolean
  Compare To Constant1 : simulink/Logic and Bit Operations/Compare To Constant  relop=>=  const=2  OutDataTypeStr=boolean
  Logical Operator : Logic  AllPortsSameDT=off  OutDataTypeStr=boolean
  Min : MinMax
  Object_Detection_Mode_idx : Constant  Value=14:14:98
  Reshape : Reshape  OutputDimensionality=Column vector (2-D)  OutputDimensions=[]
  Selector : Selector  InputPortWidth=98  IndexOptions=Index vector (port)  Indices=[1 14]  OutputSizes=1
  Selector1 : Selector  InputPortWidth=98  IndexOptions=Index vector (port)  Indices=[1 14]  OutputSizes=1
  Sensor_Enable_idx : Constant  Value=1:14:98
  2D_Sensors_Common_Signals : Outport
  wires:
  Selector/1 -> Compare To Constant/1
  Selector1/1 -> Compare To Constant1/1
  Logical Operator/1 -> Min/1
  Compare To Constant/1 -> Logical Operator/1
  Compare To Constant1/1 -> Logical Operator/2
  Object_Detection_Mode_idx/1 -> Selector1/2
  Sensor_Enable_idx/1 -> Selector/2
  Reshape/1 -> Selector/1, Selector1/1
  Sensor_Data[]/1 -> Reshape/1
  Min/1 -> Bus Creator1/1  "Sw_Enable_Discrete_Objects[0Off|1On]"
  Bus Creator1/1 -> 2D_Sensors_Common_Signals/1  "Sensors_2D_Common"

== system ASM_Traffic/Environment/Sensors/PlantModel/Object_Sensor_3D/ASMSignalCollector/Rename ==
  In1 : Inport
  Out1 : Outport  VectorParamsAs1DForOutWhenUnconnected=off
  wires:
  In1/1 -> Out1/1

== system ASM_Traffic/Environment/Sensors/PlantModel/Object_Sensor_3D/ASMSignalCollector/Rename1 ==
  In1 : Inport
  Out1 : Outport  VectorParamsAs1DForOutWhenUnconnected=off
  wires:
  In1/1 -> Out1/1

== system ASM_Traffic/Environment/Sensors/PlantModel/Object_Sensor_3D/ASMSignalCollector/Rename2 ==
  In1 : Inport
  Out1 : Outport  VectorParamsAs1DForOutWhenUnconnected=off
  wires:
  In1/1 -> Out1/1

== system ASM_Traffic/Environment/Sensors/PlantModel/Object_Sensor_3D/ASMSignalCollector/Rename3 ==
  In1 : Inport
  Out1 : Outport  VectorParamsAs1DForOutWhenUnconnected=off
  wires:
  In1/1 -> Out1/1

== system ASM_Traffic/Environment/Sensors/PlantModel/Object_Sensor_3D/ASMSignalCollector/Rename4 ==
  In1 : Inport
  Out1 : Outport  VectorParamsAs1DForOutWhenUnconnected=off
  wires:
  In1/1 -> Out1/1

== system ASM_Traffic/Environment/Sensors/PlantModel/Object_Sensor_3D/ASMSignalCollector/Rename5 ==
  In1 : Inport
  Out1 : Outport  VectorParamsAs1DForOutWhenUnconnected=off
  wires:
  In1/1 -> Out1/1

== system ASM_Traffic/Environment/Sensors/PlantModel/Object_Sensor_3D/ASMSignalCollector/Rename6 ==
  In1 : Inport
  Out1 : Outport  VectorParamsAs1DForOutWhenUnconnected=off
  wires:
  In1/1 -> Out1/1

== system ASM_Traffic/Environment/Sensors/PlantModel/Object_Sensor_3D/ASMSignalCollector/Rename7 ==
  In1 : Inport
  Out1 : Outport  VectorParamsAs1DForOutWhenUnconnected=off
  wires:
  In1/1 -> Out1/1

== system ASM_Traffic/Environment/Sensors/PlantModel/Object_Sensor_3D/ASMSignalCollector/Rename8 ==
  In1 : Inport
  Out1 : Outport  VectorParamsAs1DForOutWhenUnconnected=off
  wires:
  In1/1 -> Out1/1

== system ASM_Traffic/Environment/Sensors/PlantModel/Object_Sensor_3D/ASMSignalCollector/Sensor_1_Info ==
  Sensor_Info : Inport
  Sfcn_Status : Inport  Port=2
  Bus Creator : BusCreator  Inputs=5
  Bus Selector : BusSelector  OutputSignals=Flag_Object_In_Scope[0Out|1In],Flag_Sensor_Apex_In_Object[0Out|1In]
  Bus Selector1 : BusSelector  OutputSignals=ObjectSensor3D_Sfcn_State[],ObjectSensor3D_Data_Valid[0|1],Flag_Sensor_Init_Ready[0|1]
  Info : Outport  VectorParamsAs1DForOutWhenUnconnected=off
  wires:
  Bus Creator/1 -> Info/1
  Bus Selector1/3 -> Bus Creator/5  "<Flag_Sensor_Init_Ready[0|1]>"
  Bus Selector1/2 -> Bus Creator/4  "<ObjectSensor3D_Data_Valid[0|1]>"
  Bus Selector1/1 -> Bus Creator/3  "<ObjectSensor3D_Sfcn_State[]>"
  Bus Selector/2 -> Bus Creator/2  "<Flag_Sensor_Apex_In_Object[0Out|1In]>"
  Bus Selector/1 -> Bus Creator/1  "<Flag_Object_In_Scope[0Out|1In]>"
  Sfcn_Status/1 -> Bus Selector1/1
  Sensor_Info/1 -> Bus Selector/1

== system ASM_Traffic/Environment/Sensors/PlantModel/Object_Sensor_3D/ASMSignalCollector/Sensor_2_Info ==
  Sensor_Info : Inport
  Sensor_Status : Inport  Port=2
  Bus Creator : BusCreator  Inputs=5
  Bus Selector : BusSelector  OutputSignals=Flag_Object_In_Scope[0Out|1In],Flag_Sensor_Apex_In_Object[0Out|1In]
  Bus Selector1 : BusSelector  OutputSignals=ObjectSensor3D_Sfcn_State[],ObjectSensor3D_Data_Valid[0|1],Flag_Sensor_Init_Ready[0|1]
  Info : Outport  VectorParamsAs1DForOutWhenUnconnected=off
  wires:
  Bus Creator/1 -> Info/1
  Bus Selector1/3 -> Bus Creator/5  "<Flag_Sensor_Init_Ready[0|1]>"
  Bus Selector1/2 -> Bus Creator/4  "<ObjectSensor3D_Data_Valid[0|1]>"
  Bus Selector1/1 -> Bus Creator/3  "<ObjectSensor3D_Sfcn_State[]>"
  Bus Selector/2 -> Bus Creator/2  "<Flag_Sensor_Apex_In_Object[0Out|1In]>"
  Bus Selector/1 -> Bus Creator/1  "<Flag_Object_In_Scope[0Out|1In]>"
  Sensor_Status/1 -> Bus Selector1/1
  Sensor_Info/1 -> Bus Selector/1

== system ASM_Traffic/Environment/Sensors/PlantModel/Object_Sensor_3D/ASMSignalCollector/Sensor_3_Info ==
  Sensor_Info : Inport
  Sensor_Status : Inport  Port=2
  Bus Creator : BusCreator  Inputs=5
  Bus Selector : BusSelector  OutputSignals=Flag_Object_In_Scope[0Out|1In],Flag_Sensor_Apex_In_Object[0Out|1In]
  Bus Selector1 : BusSelector  OutputSignals=ObjectSensor3D_Sfcn_State[],ObjectSensor3D_Data_Valid[0|1],Flag_Sensor_Init_Ready[0|1]
  Info : Outport  VectorParamsAs1DForOutWhenUnconnected=off
  wires:
  Bus Creator/1 -> Info/1
  Bus Selector1/3 -> Bus Creator/5  "<Flag_Sensor_Init_Ready[0|1]>"
  Bus Selector1/2 -> Bus Creator/4  "<ObjectSensor3D_Data_Valid[0|1]>"
  Bus Selector1/1 -> Bus Creator/3  "<ObjectSensor3D_Sfcn_State[]>"
  Bus Selector/2 -> Bus Creator/2  "<Flag_Sensor_Apex_In_Object[0Out|1In]>"
  Bus Selector/1 -> Bus Creator/1  "<Flag_Object_In_Scope[0Out|1In]>"
  Sensor_Status/1 -> Bus Selector1/1
  Sensor_Info/1 -> Bus Selector/1

== system ASM_Traffic/Environment/Sensors/PlantModel/Object_Sensor_3D/CustomPoints/Sensor1 ==
  Enable[0|1] : Inport
  SensorMapping_Data[] : Inport  Port=2
  SensorData[] : Inport  Port=3
  CustomPoints : Subsystem
  CustomPointsOutput : Subsystem
  Demux : Demux
  CustomPoints_Signals[] : Outport  VectorParamsAs1DForOutWhenUnconnected=off
  wires:
  CustomPointsOutput/1(CustomPoints_Signals_Out[]) -> CustomPoints_Signals[]/1
  CustomPoints/1(CustomPoint_Signals[]) -> CustomPointsOutput/5(CustomPoints_Signals_In[])
  Enable[0|1]/1 -> CustomPointsOutput/1(SensorSchedulingEnable[0|1])
  Demux/3 -> CustomPointsOutput/4(DelayPulse[0|1])
  Demux/2 -> CustomPointsOutput/3(SensorEnable[0|1]), CustomPoints/Enable
  Demux/1 -> CustomPointsOutput/2(SensorActive[0|1])
  Demux/4 -> CustomPoints/1(Sensor_Idx[])
  SensorData[]/1 -> CustomPoints/2(Sensor_Data[])
  SensorMapping_Data[]/1 -> Demux/1

== system ASM_Traffic/Environment/Sensors/PlantModel/Object_Sensor_3D/CustomPoints/Sensor2 ==
  Enable[0|1] : Inport
  SensorMapping_Data[] : Inport  Port=2
  SensorData[] : Inport  Port=3
  CustomPoints : Subsystem
  CustomPointsOutput : Subsystem
  Demux : Demux
  CustomPoints_Signals[] : Outport  VectorParamsAs1DForOutWhenUnconnected=off
  wires:
  Demux/3 -> CustomPointsOutput/4(DelayPulse[0|1])
  Demux/2 -> CustomPoints/Enable, CustomPointsOutput/3(SensorEnable[0|1])
  CustomPointsOutput/1(CustomPoints_Signals_Out[]) -> CustomPoints_Signals[]/1
  CustomPoints/1(CustomPoint_Signals[]) -> CustomPointsOutput/5(CustomPoint_Signals_In[])
  Demux/1 -> CustomPointsOutput/2(SensorActive[0|1])
  Demux/4 -> CustomPoints/1(Sensor_Idx[])
  SensorData[]/1 -> CustomPoints/2(Sensor_Data[])
  Enable[0|1]/1 -> CustomPointsOutput/1(SensorSchedulingEnable[0|1])
  SensorMapping_Data[]/1 -> Demux/1

== system ASM_Traffic/Environment/Sensors/PlantModel/Object_Sensor_3D/CustomPoints/Sensor3 ==
  Enable[0|1] : Inport
  SensorMapping_Data[] : Inport  Port=2
  SensorData[] : Inport  Port=3
  CustomPoints : Subsystem
  CustomPointsOutput : Subsystem
  Demux : Demux
  CustomPoints_Signals[] : Outport  VectorParamsAs1DForOutWhenUnconnected=off
  wires:
  Demux/3 -> CustomPointsOutput/4(DelayPulse[0|1])
  Demux/2 -> CustomPoints/Enable, CustomPointsOutput/3(SensorEnable[0|1])
  Demux/1 -> CustomPointsOutput/2(SensorActive[0|1])
  CustomPoints/1(CustomPoint_Signals[]) -> CustomPointsOutput/5(CustomPoints_Signals_In[])
  CustomPointsOutput/1(CustomPoints_Signals_Out[]) -> CustomPoints_Signals[]/1
  Enable[0|1]/1 -> CustomPointsOutput/1(SensorSchedulingEnable[0|1])
  Demux/4 -> CustomPoints/1(Sensor_Idx[])
  SensorData[]/1 -> CustomPoints/2(Sensor_Data[])
  SensorMapping_Data[]/1 -> Demux/1

== system ASM_Traffic/Environment/Sensors/PlantModel/Object_Sensor_3D/ObjectData/BoundingBoxData_CoorSys_E ==
  Traffic_Signals : Inport
  Road_Signals : Inport  Port=2
  Sensor1_Signals[] : Inport  Port=3
  Sensor2_Signals[] : Inport  Port=4
  Sensor3_Signals[] : Inport  Port=5
  BoundingBoxData_CoorSys_E : Subsystem
  Unique_Signals_Sorted : Subsystem
  avoid_incomplete_trace2source : Subsystem
  avoid_incomplete_trace2source1 : Subsystem
  tag scope: ASMBUS_Environment_Traffic_3DObjSensors_Boundingboxes=scoped
  wires:
  avoid_incomplete_trace2source1/1(Out1) -> BoundingBoxData_CoorSys_E/2(Object_Type[])
  avoid_incomplete_trace2source/1(Out1) -> BoundingBoxData_CoorSys_E/1(Object_ID[])
  Unique_Signals_Sorted/2(Object_Type[]) -> avoid_incomplete_trace2source1/1(In1)
  Traffic_Signals/1 -> BoundingBoxData_CoorSys_E/3(Traffic_Signals)
  Unique_Signals_Sorted/1(Object_ID[]) -> avoid_incomplete_trace2source/1(In1)
  Sensor1_Signals[]/1 -> Unique_Signals_Sorted/1(Sensor1_Signals[])
  Road_Signals/1 -> BoundingBoxData_CoorSys_E/4(Road_Signals)
  Sensor2_Signals[]/1 -> Unique_Signals_Sorted/2(Sensor2_Signals[])
  Sensor3_Signals[]/1 -> Unique_Signals_Sorted/3(Sensor3_Signals[])
  BoundingBoxData_CoorSys_E/1(Boundingboxes) -> [ASMBUS_Environment_Traffic_3DObjSensors_Boundingboxes]

== system ASM_Traffic/Environment/Sensors/PlantModel/Object_Sensor_3D/ObjectData/Sensor1 ==
  Object_ID[] : Inport
  Object_Type[] : Inport  Port=2
  Traffic_Signals : Inport  Port=3
  Road_Signals : Inport  Port=4
  ASMSignalCollector : Subsystem
  Bus Selector4 : BusSelector  OutputSignals=Plant.Road_TrafficFellows.Network_Item_Type_Fellows[],Plant.Road_TrafficFellows.Network_Item_Id_Fellows[],Plant.TrafficObject_Data[]
  Bus Selector5 : BusSelector  OutputSignals=Plant.Traffic_Signals_toEnvironment
  Bus Selector6 : BusSelector  OutputSignals=Plant.ObjectParameters.TrafficObjects.TrafficObject_Type_Data[]
  GetFellowPositionVector : Subsystem
  OBJECT_POSITION : ASM_Traffic_lib/Objects/OBJECT_POSITION  MaxNumFellows=MDL.Traffic.MaxNumFellows  ASMProperties=struct('Name','OBJECT_POSITION','Version','2.0','Library','ASM_Traffic_lib')  ASMInstanceName=object_position  ASMInstanceID=1
  OBJECT_PROPERTIES_BOX : ASM_Traffic_lib/Objects/OBJECT_PROPERTIES_BOX  ASMProperties=struct('Name','OBJECT_PROPERTIES_BOX','Version','2.0','Library','ASM_Traffic_lib')  ASMInstanceName=object_properties_box  ASMInstanceID=1
  Object_Custom_Values : Subsystem
  Terminator : Terminator
  Terminator1 : Terminator
  ASMSignalBus : Outport  VectorParamsAs1DForOutWhenUnconnected=off
  Object_Position[] : Outport  Port=2  VectorParamsAs1DForOutWhenUnconnected=off
  Object_Properties_Box[] : Outport  Port=3  VectorParamsAs1DForOutWhenUnconnected=off
  Object_Custom_Values[] : Outport  Port=4  VectorParamsAs1DForOutWhenUnconnected=off
  wires:
  Bus Selector5/1 -> GetFellowPositionVector/1(<FellowPositions>)  "<Traffic_Signals_toEnvironment>"
  GetFellowPositionVector/1(Pos_Fellows_MainPnt_CoorSys_E[x;y;z][m]) -> OBJECT_POSITION/2
  GetFellowPositionVector/2(Angle_Fellows[deg]) -> OBJECT_POSITION/3
  ASMSignalCollector/1(ASMSignalBus) -> ASMSignalBus/1
  Object_Custom_Values/1(Object_Custom_Values[]) -> Object_Custom_Values[]/1, ASMSignalCollector/3(Object_Custom_Values)  "Object_Custom_Values"
  Bus Selector6/1 -> OBJECT_PROPERTIES_BOX/2, Object_Custom_Values/2(TrafficObject_Type_Data[])  "<TrafficObject_Type_Data[]>"
  Traffic_Signals/1 -> Bus Selector6/1, Bus Selector5/1
  Bus Selector4/3 -> OBJECT_POSITION/6  "<TrafficObject_Data[]>"
  Bus Selector4/2 -> OBJECT_POSITION/5  "<Network_Item_Id_Fellows[]>"
  Bus Selector4/1 -> OBJECT_POSITION/4  "<Network_Item_Type_Fellows[]>"
  Road_Signals/1 -> Bus Selector4/1
  OBJECT_PROPERTIES_BOX/2 -> Object_Properties_Box[]/1, ASMSignalCollector/2(Object_Properties_Box)
  Object_Type[]/1 -> OBJECT_PROPERTIES_BOX/1, Object_Custom_Values/1(TrafficObject_Type[])
  OBJECT_PROPERTIES_BOX/1 -> Terminator1/1  "Properties_Box"
  Object_ID[]/1 -> OBJECT_POSITION/1
  OBJECT_POSITION/1 -> Terminator/1  "Positions"
  OBJECT_POSITION/2 -> Object_Position[]/1, ASMSignalCollector/1(Object_Positions)
